simulink model "Stabilizer_QDrone_048378_OF_Ready"  (R2019a)
settings: Solver=ode2  StartTime=0.0  StopTime=inf  FixedStep=0.001  RelTol=1e-3  EnableMultiTasking=on
InitFcn:
  | addpath(fullfile(fileparts(get_param('Stabilizer_QDrone_048378_OF_Ready','FileName')),'optical_flow'));
model workspace (MAT data in the model file):
  MCOS : class17 (value not decoded)
  video_step_size = 0.06
undefined symbols (not defined in the file): datetime, gcbh, HIL, JPEG, m, OpticalFlow_, qc_get_step_size, QDrone_, saved_data, Stabilizer_, video_display_show
libraries: quarc_library x33, simulink_extras x5, simulink x4
(part 2 of 2)

== matlab function Stabilizer_QDrone_048378_OF_Ready/PHYSICAL PLANT w// LINEAR THRUST/roll and pitch approximation from accelerometer ==
  data: roll_acc output; pitch_acc output; acc_body input
function [roll_acc, pitch_acc]   = fcn(acc_body)
%#eml
n = norm(acc_body,2);
if n>eps
    acc_body = acc_body/n; 
else
    acc_body = [0 0 1]';
end

roll_acc = atan2(acc_body(2),acc_body(3));
pitch_acc = atan2( -acc_body(1), acc_body(2)*sin(roll_acc)+acc_body(3)*cos(roll_acc));

== matlab function Stabilizer_QDrone_048378_OF_Ready/STABILIZER - QDRONE/Optical Flow Monitor/Optical Flow ==
  data: image input; y output; fresh input; t input; rgb output
function [y,rgb]=run(image,fresh,t)
%#codegen
y=qdrone_of_step(image,fresh,t,false);
rgb=qdrone_of_overlay(image,y);
end

== matlab function Stabilizer_QDrone_048378_OF_Ready/Communication/Detect Communication loss/MATLAB Function ==
  settings: updateMethod=DISCRETE
  data: time input; stream_connection_loss output; state input; error input; ms_time input; data_loss output
function [stream_connection_loss , data_loss] = fcn(time, state, error, ms_time)
% signals(1) = throttle
% signals(2) = arm

persistent ms_time_prev
    if isempty(ms_time_prev)
        ms_time_prev = 0;
    end

stream_connection_loss = 0;
data_loss = 0;
if time > 3
    if ((state ~= 2)&&(error < 0))
        % stream connection is not established correctly
        stream_connection_loss = 1;
    end

    if (ms_time == ms_time_prev)
        % data is stale
        data_loss = 1;
    end
end

ms_time_prev = ms_time;

== matlab function Stabilizer_QDrone_048378_OF_Ready/PHYSICAL PLANT w// LINEAR THRUST/Red - Low Voltage Green - Armed Blue - Disarmed/MATLAB Function LED Color Assignment ==
  data: arm input; value output; low_battery input
function value = fcn(arm, low_battery)

if low_battery
    value = 1;
elseif arm
    value = 2;
else 
    value = 3;
end
